simulink model "dsPIC_33f_Explorer16"  (Simulink 7.6)
settings: Solver=FixedStepDiscrete  StartTime=0.0  StopTime=10.0  FixedStep=.005  RelTol=1e-3
undefined symbols (not defined in the file or in its folder): ANmax
libraries: dsPICdrivers x9, simulink x4
settings Model: Creator=Lubin  LastModifiedBy=Justin
settings OptimizationCC: InlineParams=on  InlineInvariantSignals=on  StateBitsets=on  DataBitsets=on  UseTempVars=on  ZeroExternalMemoryAtStartup=off  ZeroInternalMemoryAtStartup=off  OptimizeModelRefInitCode=on  LifeSpan=1
settings DebuggingCC: SaveWithParameterizedLinksMsg=none  SignalResolutionControl=TryResolveAllWithWarning  StrictBusMsg=Warning
settings HardwareCC: ProdBitPerInt=16  ProdEndianess=LittleEndian  ProdWordSize=16  ProdHWDeviceType=16-bit Generic  TargetHWDeviceType=32-bit Generic
settings RTWCC: SystemTargetFile=dspic.tlc  MakeCommand=make_CreateMPLAB  TemplateMakefile=dspic_pic30_gcc.tmf  PostCodeGenCommand=dsPIC_Compile()  Description=Embedded Target for Microchip dsPIC (real-time)  GenerateReport=on  ProcessScript=dspic_make_rtw_hook  IncludeHyperlinkInReport=on  LaunchReport=on
settings CodeAppCC: IgnoreCustomStorageClasses=off
settings STFCustomTargetCC: IncludeMdlTerminateFcn=off  CombineOutputUpdateFcns=on  SuppressErrorStatus=on  ERTCustomFileBanners=on  SupportContinuousTime=off  SupportNonInlinedSFcns=off  CPPClassGenCompliant=on  SystemTargetFile=dspic.tlc
settings ERTTargetCC: MultiwordLength=2048  ParMdlRefBuildCompliant=off  CompOptLevelCompliant=off  IncludeMdlTerminateFcn=off  SuppressErrorStatus=on  ERTFirstTimeCompliant=off  ModelStepFunctionPrototypeControlCompliant=off  InlinedParameterPlacement=NonHierarchical  ERTSrcFileBannerTemplate=dsPIC_code_template.cgt  ERTHdrFileBannerTemplate=dsPIC_code_template.cgt  ERTDataSrcFileTemplate=dsPIC_code_template.cgt  ERTDataHdrFileTemplate=dsPIC_code_template.cgt  ERTCustomFileTemplate=dsPIC_main.tlc  ConvertIfToSwitch=off
settings CustomProperty: DataType=string  Value=C:\PROGRA~1\MATLAB\R2010b\bin\win32\gmake

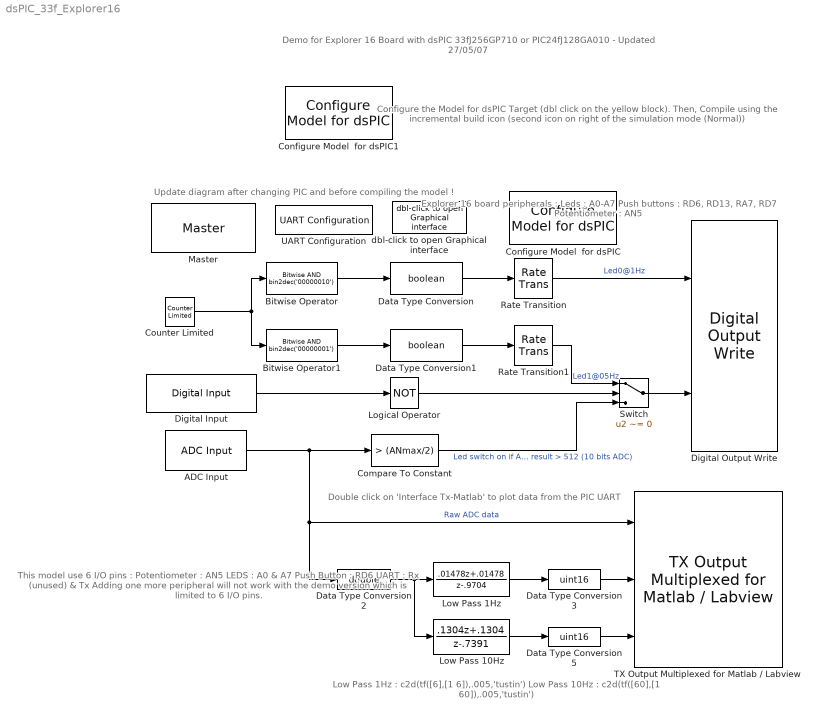
== system dsPIC_33f_Explorer16 ==
  note: Low Pass 1Hz : c2d(tf([6],[1 6]),.005,'tustin')
      | Low Pass 10Hz : c2d(tf([60],[1 60]),.005,'tustin')
  note: Demo for Explorer 16 Board with dsPIC 33fJ256GP710 or PIC24fJ128GA010 - Updated 27/05/07
  note: Explorer 16 board peripherals :
      | Leds : A0-A7
      | Push buttons : RD6, RD13, RA7, RD7
      | Potentiometer : AN5
  note: This model use 6 I/O pins :
      | Potentiometer : AN5
      | LEDS : A0 & A7
      | Push Button : RD6
      | UART : Rx (unused) & Tx
      | Adding one more peripheral will not
      | work with the demo version which is
      | limited to 6 I/O pins.
  note: Double click on 'Interface Tx-Matlab' to plot data from the PIC UART
  note: Update diagram after changing PIC and before compiling the model !
  note: Configure the Model for dsPIC Target (dbl click on the yellow block).
      | Then, Compile using the incremental build icon
      | (second icon on right of the simulation mode (Normal))
  ADC Input : dsPICdrivers/Peripheral I//O/ADC Input  Tag=dsPIC_ADC  Priority=5  ADC_TYPE=10 bits  ADC_MODE=Continuous sampling & get last channel value  NbrSampleStep=1  VoltRefpopup="AVdd  -  AVss"  OutFormatBitspopup=0000 00dd dddd dddd : Integer  InterruptPriority=6  ANCHANNELS=[5]  MaxName=ANmax = 1023  Rin=5e6  ADCS=12  SAMC=31  Temperature=25  DMAChannel=0  SampleTime=.005  Status="OK  |  Tsmp=5.038e-006 |  T/Channel=6.988e-006 |  Tall=6.988e-006"  SSRC=auto convert
  Bitwise Operator : simulink/Logic and Bit Operations/Bitwise Operator  logicop=AND  UseBitMask=on  BitMask=bin2dec('00000010')  BitMaskRealWorld=Stored Integer
  Bitwise Operator1 : simulink/Logic and Bit Operations/Bitwise Operator  logicop=AND  UseBitMask=on  BitMask=bin2dec('00000001')  BitMaskRealWorld=Stored Integer
  Compare To Constant : simulink/Logic and Bit Operations/Compare To Constant  SystemSampleTime=-1  relop=>  const=(ANmax/2)  LogicOutDataTypeMode=boolean  ZeroCross=off
  Configure Model  for dsPIC : dsPICdrivers/Simulink Configuration/Configure Model  for dsPIC
  Configure Model  for dsPIC1 : dsPICdrivers/Simulink Configuration/Configure Model  for dsPIC
  Counter Limited : simulink/Sources/Counter Limited  SystemSampleTime=-1  uplimit=3  tsamp=.25
  Data Type Conversion : DataTypeConversion  OutDataTypeStr=boolean
  Data Type Conversion1 : DataTypeConversion  OutDataTypeStr=boolean
  Data Type Conversion2 : DataTypeConversion  OutDataTypeStr=double
  Data Type Conversion3 : DataTypeConversion  OutDataTypeStr=uint16
  Data Type Conversion5 : DataTypeConversion  OutDataTypeStr=uint16
  Digital Input : dsPICdrivers/Digital I//O/Digital Input  Tag=dsPIC_Digital_Input  PORT=D  Pin=[6]  SampleTime=-1  OrderingInOutPopup=None
  Digital Output Write : dsPICdrivers/Digital I//O/Digital Output Write  Tag=dsPIC_Digital_Output  Priority=5  PORT=A  Pin="[0  7 ]"  Simultaneous=off  OrderingInOutPopup=None
  Logical Operator : Logic  Operator=NOT  AllPortsSameDT=off  OutDataTypeStr=boolean
  Low Pass 10Hz : DiscreteTransferFcn  Numerator=[.1304 .1304]  Denominator=[1 -.7391]  SampleTime=-1
  Low Pass 1Hz : DiscreteTransferFcn  Numerator=[.01478 .01478]  Denominator=[1 -.9704]  SampleTime=-1
  Master : dsPICdrivers/Master  Tag=dsPIC_MASTER  Priority=1  TimeStepType=Timer1  picType=33fJ256GP710  fcy=40000000  Quartz_33f=8e6  PLLActive_33f=on  fcyDesired_33f=40000000  tmr1="[1  19999  0]"  tmr1Info="Time Step : 0.005  ;   Error : 0%  PR1=24999"  tmr2345="[0  0  0  0  0  0  0  0]"  tmr2345cfg=[-1 -1 -1 -1 -1 -1 -1 -1]  IOautoConf=on  typePort="[ 10   0   0   0   0   0   0  10   0   0   0   0   0   0   0   0   0   0   0   0   0   8   0   0   0   0   0   0   0   0   0   0   0   0   0   0   0   0   0   0   0   0   0   0   0   0   0   0   0   0   0   0   0   0   9   0   0   0   0   0   0   0   0   0   0   0   0   0   0   0   0   0   0   0   0   0   0   0   0   0   0   0   0   0   4   5   0   0   0   0   0   0   0   0   0   0   0   0   0   0   0   0   0   0   0   0   0   0   0   0   0   0 ]"  TRIS="[ 65406  65535  65535  65535  65535  65535  65535 ]"  ADPCFG=8388608  MasterBusyPort=None  MasterOverloadPort=None  FOSC=Quartz (XT - HS)  ClockSwitchMonitor=Both disabled  TempProtection_33f=TEMP_ON  FPBOR=<empty>  PWRT=disable  MCLR=<empty>  ICD=ICS_PGD1  JTAGEN=JTAGEN_OFF  PowerSave=off  OverrideFcy=off  NewFcy=1e6  PR2345="[65535  65535  65535  65535  65535  65535  65535  65535]"
  Rate Transition : RateTransition
  Rate Transition1 : RateTransition
  Switch : Switch  Criteria=u2 ~= 0
  TX Output Multiplexed for Matlab / Labview : dsPICdrivers/Serial PORT/TX Output Multiplexed for Matlab // Labview  Tag=dsPIC_TX_Multiplexed  Priority=5  UART=2  CleverSpreadingChk=on  CleverSpreading=1  CHANNEL=[0 1 2]  CHANNELBLOCKED=[]  CHANNELBLOCKED_BITEWISE=0  Status=OK
  UART Configuration : dsPICdrivers/Serial PORT/UART Configuration  Tag=dsPIC_config_UART  Priority=2  UART=2  proposed_BAUD=19200  ALT_TX_RX=off  InterruptTxWhen=When Transmit Buffer is empty  TXInterruptPri=7  TxBufferSize=32  TXEN=on  InterruptRxWhen=When Receive Buffer is full (contain 4 characters)  RXInterruptPri=1  RxBufferSize=32  BAUD=19200  UxBRG=129  Info="UxBRG = 129   ||  Real Baud : 19231   ||  % error : 0.16026  ||  max 9.6154 Bytes / Step"  RealBaud=0
  dbl-click to open Graphical interface : dsPICdrivers/Serial PORT/dbl-click to open Graphical interface  Nothing=0
  wires:
  Counter Limited/1 -> Bitwise Operator/1, Bitwise Operator1/1
  ADC Input/1 -> Compare To Constant/1, TX Output Multiplexed for Matlab / Labview/1, Data Type Conversion2/1  "Raw ADC data"
  Bitwise Operator1/1 -> Data Type Conversion1/1
  Bitwise Operator/1 -> Data Type Conversion/1
  Rate Transition/1 -> Digital Output Write/1  "Led0@1Hz"
  Data Type Conversion/1 -> Rate Transition/1
  Data Type Conversion1/1 -> Rate Transition1/1
  Data Type Conversion2/1 -> Low Pass 1Hz/1, Low Pass 10Hz/1
  Low Pass 1Hz/1 -> Data Type Conversion3/1
  Data Type Conversion3/1 -> TX Output Multiplexed for Matlab / Labview/2
  Low Pass 10Hz/1 -> Data Type Conversion5/1
  Data Type Conversion5/1 -> TX Output Multiplexed for Matlab / Labview/3
  Digital Input/1 -> Logical Operator/1
  Compare To Constant/1 -> Switch/3  "Led switch on if AN result > 512 (10 bits ADC)"
  Rate Transition1/1 -> Switch/1  "Led1@05Hz"
  Switch/1 -> Digital Output Write/2
  Logical Operator/1 -> Switch/2
